simulink model "ModelSilnika_MiI2012"  (R2024b)
settings: Solver=FixedStepAuto  StartTime=0.0  StopTime=200  FixedStep=0.1  RelTol=1e-3  EnableMultiTasking=on
libraries: SignalEditorBlockLib x3, simulink x1
settings Model: Creator=Milo  LastModifiedBy=Milo
settings SolverCC: AlgebraicLoopSolver=TrustRegion
settings DataIOCC: LimitDataPoints=on  SaveFormat=Array  SignalLoggingSaveFormat=ModelDataLogs  ReturnWorkspaceOutputs=off
settings OptimizationCC: InitFltsAndDblsToZero=on  LifeSpan=inf
settings DebuggingCC: SaveWithParameterizedLinksMsg=none  UnderspecifiedInitializationDetection=Classic  MergeDetectMultiDrivingBlocksExec=none  SignalResolutionControl=TryResolveAllWithWarning  SolverPrmCheckMsg=warning  MultiTaskDSMMsg=warning  MultiTaskCondExecSysMsg=none  FcnCallInpInsideContextMsg=warning  UnconnectedInputMsg=warning  UnconnectedOutputMsg=warning  UnconnectedLineMsg=warning  SFUnexpectedBacktrackingDiag=warning  SFNoUnconditionalDefaultTransitionDiag=warning  SFExecutionAtInitializationDiag=none  ArithmeticOperatorsInVariantConditions=warning
settings HardwareCC: ProdBitPerPointer=32  ProdBitPerSizeT=32  ProdBitPerPtrDiffT=32  ProdLargestAtomicFloat=None  ProdIntDivRoundTo=Undefined  ProdEndianess=Unspecified  ProdWordSize=32  ProdHWDeviceType=32-bit Generic
settings ModelReferenceCC: PropagateSignalLabelsOutOfModel=off
settings RTWCC: GPUComputeCapability=3.5
settings CodeAppCC: StateflowObjectComments=on
settings GRTTargetCC: TargetFcnLib=ansi_tfl_tmw.mat  TargetLangStandard=C89/C90 (ANSI)  CombineOutputUpdateFcns=off  GRTInterface=on
settings ConfigComp: CovMetricSettings=dw  CovSaveCumulativeToWorkspaceVar=on  CovSaveSingleToWorkspaceVar=on

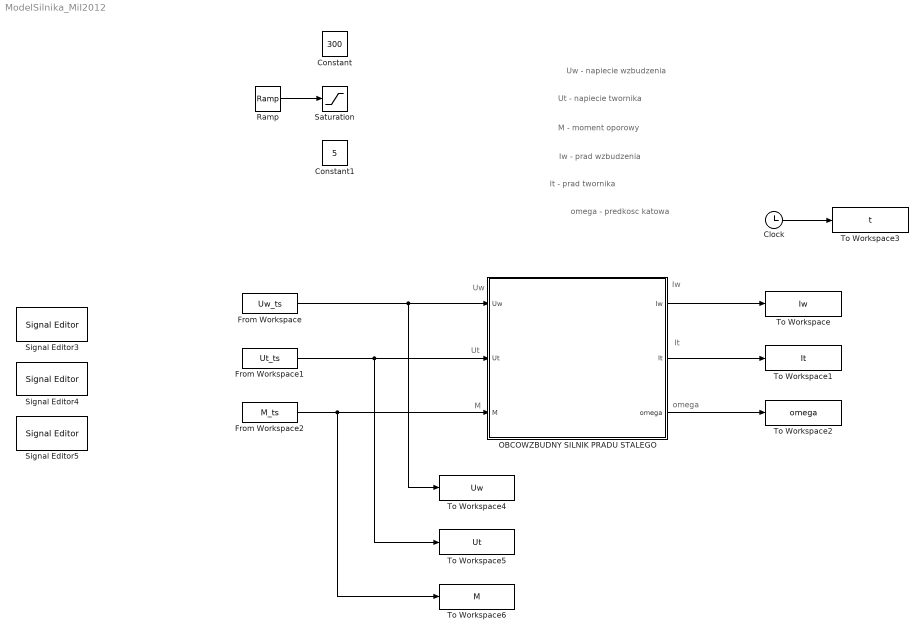
== system ModelSilnika_MiI2012 ==
  note: Uw
  note: Ut
  note: M
  note: Iw
  note: It
  note: omega
  note: Uw - napiecie wzbudzenia
  note: Ut - napiecie twornika
  note: M - moment oporowy
  note: Iw - prad wzbudzenia
  note: It - prad twornika
  note: omega - predkosc katowa
  Clock : Clock
  Constant : Constant  Value=300
  Constant1 : Constant  Value=5
  From Workspace : FromWorkspace  VariableName=Uw_ts
  From Workspace1 : FromWorkspace  VariableName=Ut_ts
  From Workspace2 : FromWorkspace  VariableName=M_ts
  OBCOWZBUDNY SILNIK PRADU STALEGO : Subsystem
      mask init:
      | [data, map]=imread('silnik.gif');
      | pic=ind2rgb(data,map);
      mask Display: image(pic)
  Ramp : simulink/Sources/Ramp  slope=15  start=0  InitialOutput=0
  Saturation : Saturate  UpperLimit=300  LowerLimit=0
  Signal Editor3 : SignalEditorBlockLib/Signal Editor  FileName=Uw.mat  ActiveScenario=Scenario  ActiveSignal=Signal 1  IsBus=off  OutputBusObjectStr=Bus: BusObject  SampleTime=0  Interpolate=off  ZeroCross=off  OutputAfterFinalValue=Setting to zero  Unit=inherit  PreserveSignalName=on  ApplySigPropsToAllScenarios=on  ApplySigPropsToAllSignals=off
  Signal Editor4 : SignalEditorBlockLib/Signal Editor  FileName=Ut.mat  ActiveScenario=Scenario  ActiveSignal=Signal 1  IsBus=off  OutputBusObjectStr=Bus: BusObject  SampleTime=0  Interpolate=off  ZeroCross=off  OutputAfterFinalValue=Setting to zero  Unit=inherit  PreserveSignalName=on  ApplySigPropsToAllScenarios=on  ApplySigPropsToAllSignals=off
  Signal Editor5 : SignalEditorBlockLib/Signal Editor  FileName=M.mat  ActiveScenario=Scenario  ActiveSignal=Signal 1  IsBus=off  OutputBusObjectStr=Bus: BusObject  SampleTime=0  Interpolate=off  ZeroCross=off  OutputAfterFinalValue=Setting to zero  Unit=inherit  PreserveSignalName=on  ApplySigPropsToAllScenarios=on  ApplySigPropsToAllSignals=off
  To Workspace : ToWorkspace  VariableName=Iw  SampleTime=-1
  To Workspace1 : ToWorkspace  VariableName=It  SampleTime=-1
  To Workspace2 : ToWorkspace  VariableName=omega  SampleTime=-1
  To Workspace3 : ToWorkspace  VariableName=t  SampleTime=-1
  To Workspace4 : ToWorkspace  VariableName=Uw  SampleTime=-1
  To Workspace5 : ToWorkspace  VariableName=Ut  SampleTime=-1
  To Workspace6 : ToWorkspace  VariableName=M  SampleTime=-1
  wires:
  Ramp/1 -> Saturation/1
  OBCOWZBUDNY SILNIK PRADU STALEGO/1(Iw) -> To Workspace/1
  OBCOWZBUDNY SILNIK PRADU STALEGO/2(It) -> To Workspace1/1
  OBCOWZBUDNY SILNIK PRADU STALEGO/3(omega) -> To Workspace2/1
  Clock/1 -> To Workspace3/1
  From Workspace/1 -> To Workspace4/1, OBCOWZBUDNY SILNIK PRADU STALEGO/1(Uw)
  From Workspace1/1 -> To Workspace5/1, OBCOWZBUDNY SILNIK PRADU STALEGO/2(Ut)
  From Workspace2/1 -> To Workspace6/1, OBCOWZBUDNY SILNIK PRADU STALEGO/3(M)

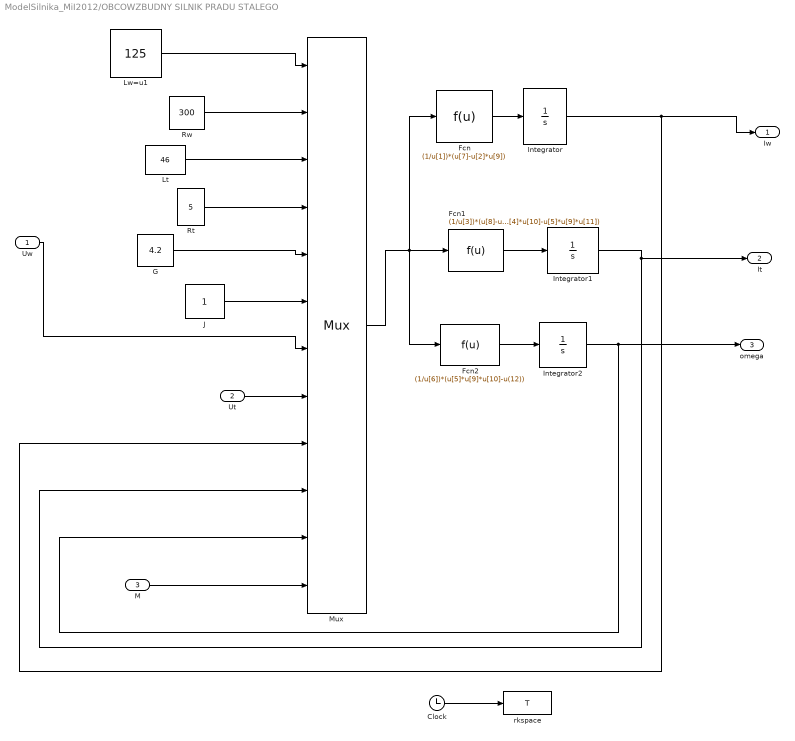
== system ModelSilnika_MiI2012/OBCOWZBUDNY SILNIK PRADU STALEGO ==
  Uw : Inport
  Ut : Inport  Port=2
  M : Inport  Port=3
  Clock : Clock
  Fcn : Fcn  Expr=(1/u[1])*(u[7]-u[2]*u[9])
  Fcn1 : Fcn  Expr=(1/u[3])*(u[8]-u[4]*u[10]-u[5]*u[9]*u[11])
  Fcn2 : Fcn  Expr=(1/u[6])*(u[5]*u[9]*u[10]-u(12))
  G : Constant  Value=4.2
  Integrator : Integrator
  Integrator1 : Integrator
  Integrator2 : Integrator
  J : Constant
  Lt : Constant  Value=46
  Lw=u1 : Constant  Value=125
  Mux : Mux  Inputs=12
  Rt : Constant  Value=5
  Rw : Constant  Value=300
  rkspace : ToWorkspace  VariableName=T  SampleTime=-1
  Iw : Outport
  It : Outport  Port=2
  omega : Outport  Port=3
  wires:
  Lw=u1/1 -> Mux/1
  Rw/1 -> Mux/2
  Lt/1 -> Mux/3
  J/1 -> Mux/6
  Fcn/1 -> Integrator/1
  Fcn1/1 -> Integrator1/1
  Rt/1 -> Mux/4
  Integrator/1 -> Mux/9, Iw/1
  Integrator1/1 -> Mux/10, It/1
  Fcn2/1 -> Integrator2/1
  Integrator2/1 -> Mux/11, omega/1
  Mux/1 -> Fcn2/1, Fcn/1, Fcn1/1
  G/1 -> Mux/5
  Clock/1 -> rkspace/1
  Uw/1 -> Mux/7
  M/1 -> Mux/12
  Ut/1 -> Mux/8
